simulink model "commhdlQPSKTxRxLoopback"  (R2025b)
settings: Solver=FixedStepDiscrete  StartTime=0.0  StopTime=0.03  RelTol=1e-3
PostLoadFcn:
  | hScopeConfig = get_param([gcs '/Receiver/QPSK Rx/Frequency and Time Synchronizer/Symbol Synchronizer/No HDL/QPSK Receiver Eye Diagram'],'ScopeConfiguration');
  | 
  | hScopeConfig.OpenAtSimulationStart = false;
  | hScopeConfig.Visible = false;
  | SamplesPerSymbol = 4;
  | %UpsamplesRx = 1;
  | clear hScopeConfig
InitFcn:
  | % RxAlign decoder latency (flat_simfix): 41 = netlist value used for HDL; set
  | % rxAlignLat = 25 in the base workspace before a model-level simulation.
  | if ~exist('rxAlignLat','var'), rxAlignLat = uint16(41); end
  | commhdlQPSKTxRxModelInit;
  | % Rate bridge: ADRV9002/Jupiter radio runs at 15.36 MHz = 2x the 7.68 MHz
  | % (4 samples/symbol @ Rsym=1.92 MHz) the QPSK Rx requires. The deployed
  | % Receiver must downsample the ADC stream by 2. UpsamplesRx=1 fed the QPSK
  | % Rx 8 sps (2x-upsampled) and broke symbol sync / the loopback bit check.
  | UpsamplesRx = 1;   %% T8 RATE FIX: rail 15.36e6 == ADC bus rate,
  | %% no ingress decimation (was 2 when the rail sat on the 7.68e6 rung)
  | UpsamplesTx = 1;
  | clear simTimingOffset;
StopFcn:
  | if exist('simTimingOffset','var')
  |   disp('Simulation completed');
  |   %QPSKTxRxVerification;
  | end
undefined symbols (not defined in the file or in its folder): Add, Config, fsym, randsrc, RandStream, Rsym, rxAlignLat, Shift
libraries: hdlsllib x141, simulink x45, dspsigops x30, dsphdlfiltering2 x6, dsphdlsigops2 x4, dsphdlmathfun2 x4, commdigbbndpm3 x4, dspmlti4 x2, commchan3 x1, commrflib2 x1, commcnvcod2 x1
(part 4 of 9)

== system commhdlQPSKTxRxLoopback/Transmitter/QPSK Tx/Bit Packetizer/Preamble Bits Generator ==
  activeFrame : Inport
  sampleCount : Inport  Port=2
  sampleCountValid : Inport  Port=3
  Compare To Constant2 : hdlsllib/Logic and Bit Operations/Compare To Constant  relop===  const=bitsPerPacket - 1  OutDataTypeStr=boolean
  Logical Operator3 : Logic  AllPortsSameDT=off  OutDataTypeStr=boolean
  Preamble Bits Store : Subsystem
  Unit Delay Enabled Synchronous : hdlsllib/Discrete/Unit Delay Enabled Synchronous  InitialCondition=0.0  SampleTime=-1
  preambleBits : Outport
  wires:
  sampleCount/1 -> Compare To Constant2/1, Preamble Bits Store/2(sampleCount)
  Logical Operator3/1 -> Unit Delay Enabled Synchronous/2
  Preamble Bits Store/1(preamble) -> preambleBits/1
  Compare To Constant2/1 -> Logical Operator3/1
  Unit Delay Enabled Synchronous/1 -> Preamble Bits Store/1(actualPreamble)
  sampleCountValid/1 -> Logical Operator3/2
  activeFrame/1 -> Unit Delay Enabled Synchronous/1

== system commhdlQPSKTxRxLoopback/TxRxComposite/Receiver/QPSK Rx/Automatic Gain Control ==
  dataIn : Inport
  validIn : Inport  Port=2
  agc_loop_gain : Inport  Port=3  OutDataTypeStr=uint32  SampleTime=1/(Rsym*SamplesPerSymbol)
  Data Type Conversion : DataTypeConversion  OutDataTypeStr=fixdt(1,16,10)  SaturateOnIntegerOverflow=off  RndMeth=Floor
  Delay{1..5} (5 alike) : Delay
  Error Detector : Subsystem
  Loop Filter : Subsystem
  Product : Product  OutDataTypeStr=Inherit: Same as first input
  dataOut : Outport
  validOut : Outport  Port=2
  wires:
  Product/1 -> Delay2/1
  Error Detector/1(err) -> Loop Filter/1(err)
  Delay1/1 -> Product/2
  Delay4/1 -> Product/1
  Delay3/1 -> validOut/1
  Delay2/1 -> dataOut/1, Error Detector/1(dataIn)
  Data Type Conversion/1 -> Delay1/1
  Loop Filter/1(gain) -> Data Type Conversion/1
  dataIn/1 -> Delay4/1
  Delay5/1 -> Delay3/1
  agc_loop_gain/1 -> Loop Filter/2(agc_loop_gain)
  validIn/1 -> Delay5/1

== system commhdlQPSKTxRxLoopback/TxRxComposite/Receiver/QPSK Rx/FEC Decoder Wrapper ==
  bitsIn : Inport
  startIn : Inport  Port=2
  endIn : Inport  Port=3
  validIn : Inport  Port=4
  skipCount : Inport  Port=5  OutDataTypeStr=uint32  SampleTime=1/(Rsym*SamplesPerSymbol)
  FecCapture : MATLAB Function  TreatAsAtomicUnit=on
  FecCounters : MATLAB Function  TreatAsAtomicUnit=on
  RxAlign : MATLAB Function  TreatAsAtomicUnit=on
  RxAlignLatency : Constant  Description=Decoder latency absorbed by RxAlign. rxAlignLat = 41 (netlist, default from InitFcn) or 25 (model simulation).  Value=rxAlignLat  OutDataTypeStr=uint16  SampleTime=Inf
  RxDeint : MATLAB Function  TreatAsAtomicUnit=on
  VitGate : Subsystem
  dataOut : Outport
  startOut : Outport  Port=2
  endOut : Outport  Port=3
  validOut : Outport  Port=4
  cnt_descr_in : Outport  Port=5
  cnt_frame_start : Outport  Port=6
  cnt_vit_reset : Outport  Port=7
  cnt_deint_valid : Outport  Port=8
  cnt_dec_bits : Outport  Port=9
  cnt_bist_start : Outport  Port=10
  cap_in : Outport  Port=11
  cap_deint : Outport  Port=12
  cap_out : Outport  Port=13
  wires:
  FecCounters/6(c6) -> cnt_bist_start/1
  FecCounters/3(c3) -> cnt_vit_reset/1
  FecCounters/2(c2) -> cnt_frame_start/1
  FecCapture/3(capOut) -> cap_out/1
  FecCapture/2(capDeint) -> cap_deint/1
  RxAlign/4(validOut) -> FecCapture/8(outValid), FecCounters/5(e5), validOut/1
  FecCapture/1(capIn) -> cap_in/1
  RxAlign/3(endOut) -> endOut/1
  bitsIn/1 -> RxDeint/1(dataIn), FecCapture/1(bitsIn)
  validIn/1 -> RxDeint/4(validIn), FecCounters/1(e1), FecCapture/2(validIn)
  FecCounters/5(c5) -> cnt_dec_bits/1
  startIn/1 -> RxDeint/2(startIn), FecCounters/2(e2), FecCapture/3(startIn)
  FecCounters/4(c4) -> cnt_deint_valid/1
  endIn/1 -> RxDeint/3(endIn)
  RxDeint/5(frameEnd) -> RxAlign/4(frameEnd)
  VitGate/1(decOut) -> RxAlign/1(decBit)
  RxDeint/1(codedPair) -> VitGate/1(pairIn), FecCapture/4(codedPair)
  FecCounters/1(c1) -> cnt_descr_in/1
  RxDeint/2(vitReset) -> VitGate/2(rstIn), FecCounters/3(e3)
  RxDeint/3(deintValid) -> VitGate/Enable, FecCounters/4(e4), RxAlign/2(deintValid), FecCapture/5(deintValid)
  skipCount/1 -> RxAlign/5(skipCount), FecCapture/7(skipCount)
  RxDeint/4(frameStart) -> RxAlign/3(frameStart)
  RxAlign/1(dataOut) -> FecCapture/6(decBit), dataOut/1
  RxAlign/2(startOut) -> FecCounters/6(e6), startOut/1
  RxAlignLatency/1 -> RxAlign/6(alignLat)

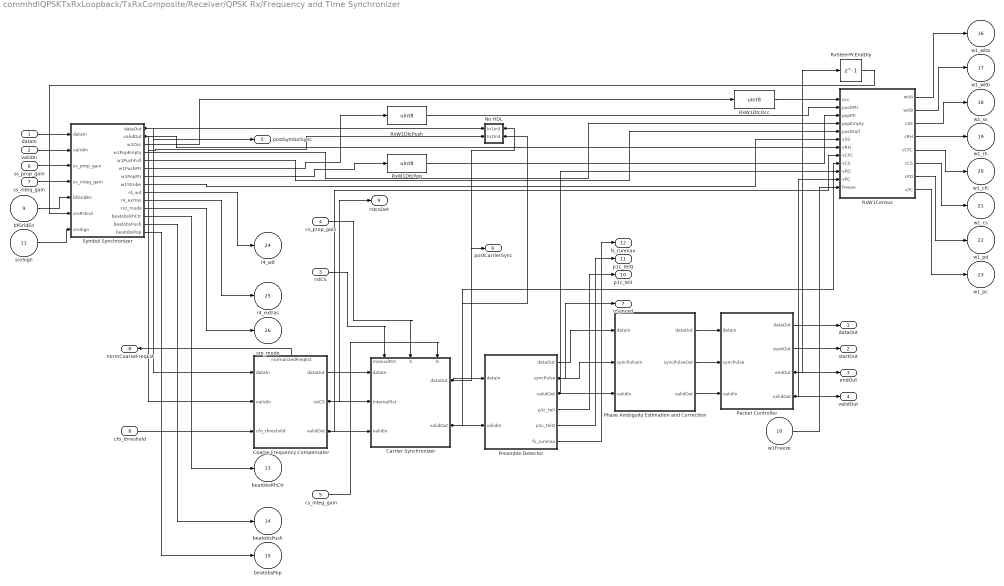
== system commhdlQPSKTxRxLoopback/TxRxComposite/Receiver/QPSK Rx/Frequency and Time Synchronizer ==
  dataIn : Inport
  validIn : Inport  Port=2
  rstCS : Inport  Port=3
  cs_prop_gain : Inport  Port=4  OutDataTypeStr=uint32  SampleTime=1/(Rsym*SamplesPerSymbol)
  cs_integ_gain : Inport  Port=5  OutDataTypeStr=uint32  SampleTime=1/(Rsym*SamplesPerSymbol)
  ss_prop_gain : Inport  Port=6  OutDataTypeStr=uint32  SampleTime=1/(Rsym*SamplesPerSymbol)
  ss_integ_gain : Inport  Port=7  OutDataTypeStr=uint32  SampleTime=1/(Rsym*SamplesPerSymbol)
  cfo_threshold : Inport  Port=8  OutDataTypeStr=uint32  SampleTime=1/(Rsym*SamplesPerSymbol)
  bfGridEn : Inport  Port=9  OutDataTypeStr=boolean
  w1Freeze : Inport  Port=10  OutDataTypeStr=boolean
  sroSign : Inport  Port=11  OutDataTypeStr=boolean
  Carrier Synchronizer : Subsystem
      settings: PortSchema="{\"entries\":[{\"content\":{\"sides\":[{\"content\":{\"connectorIds\":[\"In1\",\"In2\",\"In3\"]},\"type\":\"ConnectorPlacement.EquallySpacedRectSide\",\"uuid\":\"ee58e5dc-083a-48cb-b7f3-66ed8a15890f\"},{\"content\":{\"connectorIds\":[\"Out1\",\"Out2\"],\"side\":\"RIGHT\"},\"type\":\"ConnectorPlacement.EquallySpacedRectSide\",\"uuid\":\"6d121164-5065-4840-a82e-fa57a8e9650e\"},{\"content\":{\"connectorIds\":[\"In4\",\"In5\",\"In6\"],\"side\":\"TOP\"},\"type\":\"ConnectorPlacement.EquallySpacedRectSide\",\"uuid\":\"54d2b8e3-f516-4572-94a0-c914196ae8e4\"}]},\"type\":\"ConnectorPlacement.EquallySpacedConnector\",\"uuid\":\"0f2a6472-efd0-42ca-a030-ab436081b5e1\"}],\"packageUris\":[\"http://schema.mathworks.com/mf0/Connector/R2020b\"],\"version\":\"1.0\"}"
  Coarse Frequency Compensator : Subsystem
      settings: PortSchema="{\"entries\":[{\"content\":{\"sides\":[{\"content\":{\"connectorIds\":[\"In1\",\"In2\",\"In3\"]},\"type\":\"ConnectorPlacement.EquallySpacedRectSide\",\"uuid\":\"138aa5bd-62db-47d6-b55f-f529a6004434\"},{\"content\":{\"connectorIds\":[\"Out1\",\"Out2\",\"Out3\"],\"side\":\"RIGHT\"},\"type\":\"ConnectorPlacement.EquallySpacedRectSide\",\"uuid\":\"8e6ccec0-f736-48ab-be6d-feac886e083d\"},{\"content\":{\"connectorIds\":[\"Out4\"],\"side\":\"TOP\"},\"type\":\"ConnectorPlacement.EquallySpacedRectSide\",\"uuid\":\"d4535392-74fa-432a-a39c-b98ba26e8163\"},{\"content\":{\"side\":\"BOTTOM\"},\"type\":\"ConnectorPlacement.EquallySpacedRectSide\",\"uuid\":\"770ac6a2-7a02-4a77-858b-592982deaf6e\"}]},\"type\":\"ConnectorPlacement.EquallySpacedConnector\",\"uuid\":\"a9b944be-f88b-4ab6-a5e1-6824362eb9ca\"}],\"packageUris\":[\"http://schema.mathworks.com/mf0/Connector/R2020b\"],\"version\":\"1.0\"}"
  No HDL : Subsystem
      settings: PortSchema="{\"entries\":[{\"content\":{\"sides\":[{\"content\":{\"connectorIds\":[\"In1\",\"In2\"]},\"type\":\"ConnectorPlacement.EquallySpacedRectSide\",\"uuid\":\"df96a46d-149f-4580-adf6-e5cf26cffa9b\"},{\"content\":{\"connectorIds\":[\"In3\",\"In4\"],\"side\":\"RIGHT\"},\"type\":\"ConnectorPlacement.EquallySpacedRectSide\",\"uuid\":\"1c46d09c-cb37-4618-ac4e-e5ef50df41fb\"},{\"content\":{\"connectorIds\":[],\"side\":\"TOP\"},\"type\":\"ConnectorPlacement.EquallySpacedRectSide\",\"uuid\":\"7fe62300-46d7-4234-a31d-eecffed4f6e6\"},{\"content\":{\"connectorIds\":[],\"side\":\"BOTTOM\"},\"type\":\"ConnectorPlacement.EquallySpacedRectSide\",\"uuid\":\"05ecd563-28f5-4cfd-b718-5032a7458763\"}]},\"type\":\"ConnectorPlacement.EquallySpacedConnector\",\"uuid\":\"4b3d5859-a469-4389-9e5d-e5f07416a9a1\"}],\"packageUris\":[\"http://schema.mathworks.com/mf0/Connector/R2020b\"],\"version\":\"1.0\"}"
  Packet Controller : Subsystem
  Phase Ambiguity Estimation and Correction : Subsystem
  Preamble Detector : Subsystem
  RxSteerPcEndDly : Delay  DelayLength=1
  RxW1Census : MATLAB Function  TreatAsAtomicUnit=on
  RxW1DtcOcc : DataTypeConversion  OutDataTypeStr=uint8  ConvertRealWorld=Stored Integer (SI)  SaturateOnIntegerOverflow=off  RndMeth=Floor
  RxW1DtcPop : DataTypeConversion  OutDataTypeStr=uint8  ConvertRealWorld=Stored Integer (SI)  SaturateOnIntegerOverflow=off  RndMeth=Floor
  RxW1DtcPush : DataTypeConversion  OutDataTypeStr=uint8  ConvertRealWorld=Stored Integer (SI)  SaturateOnIntegerOverflow=off  RndMeth=Floor
  Symbol Synchronizer : Subsystem
  dataOut : Outport
  startOut : Outport  Port=2
  endOut : Outport  Port=3
  validOut : Outport  Port=4
  postSymbolSync : Outport  Port=5
  postCarrierSync : Outport  Port=6
  nSynced : Outport  Port=7
  normCoarseFreqEst : Outport  Port=8
  rstcsDet : Outport  Port=9
  p1c_telI : Outport  Port=10
  p1c_telQ : Outport  Port=11
  fs_runmax : Outport  Port=12
  beatobsRhCtr : Outport  Port=13
  beatobsPush : Outport  Port=14
  beatobsPop : Outport  Port=15
  w1_wita : Outport  Port=16
  w1_witb : Outport  Port=17
  w1_ss : Outport  Port=18
  w1_rh : Outport  Port=19
  w1_cfc : Outport  Port=20
  w1_cs : Outport  Port=21
  w1_pd : Outport  Port=22
  w1_pc : Outport  Port=23
  r4_wit : Outport  Port=24
  r4_extras : Outport  Port=25
  sro_mode : Outport  Port=26
  wires:
  RxW1Census/6(cCS) -> w1_cs/1
  RxSteerPcEndDly/1 -> Symbol Synchronizer/6(sroPcEnd)
  w1Freeze/1 -> RxW1Census/12(freeze)
  RxW1DtcOcc/1 -> RxW1Census/1(occ)
  Phase Ambiguity Estimation and Correction/2(syncPulseOut) -> Packet Controller/2(syncPulse)
  Phase Ambiguity Estimation and Correction/1(dataOut) -> Packet Controller/1(dataIn)
  RxW1Census/8(cPC) -> w1_pc/1
  Preamble Detector/6(fs_runmax) -> fs_runmax/1
  Preamble Detector/4(p1c_telI) -> p1c_telI/1
  Preamble Detector/1(dataOut) -> Phase Ambiguity Estimation and Correction/1(dataIn)
  RxW1DtcPush/1 -> RxW1Census/2(pushPtr)
  Symbol Synchronizer/7(w1PopPtr) -> RxW1DtcPop/1
  Symbol Synchronizer/5(w1PushFull) -> RxW1Census/5(pushFull)
  RxW1Census/1(witA) -> w1_wita/1
  cs_prop_gain/1 -> Carrier Synchronizer/5(cs_prop_gain)
  Symbol Synchronizer/4(w1PopEmpty) -> RxW1Census/4(popEmpty)
  RxW1Census/7(cPD) -> w1_pd/1
  Phase Ambiguity Estimation and Correction/3(validOut) -> Packet Controller/3(validIn)
  Symbol Synchronizer/2(validOut) -> Coarse Frequency Compensator/2(validIn), RxW1Census/7(vRH), No HDL/2(In2)
  Packet Controller/2(startOut) -> startOut/1
  sroSign/1 -> Symbol Synchronizer/7(sroSign)
  bfGridEn/1 -> Symbol Synchronizer/5(bfGridEn)
  Carrier Synchronizer/2(validOut) -> Preamble Detector/2(validIn), No HDL/4(In4), RxW1Census/9(vCS)
  cfo_threshold/1 -> Coarse Frequency Compensator/3(cfo_threshold)
  RxW1DtcPop/1 -> RxW1Census/3(popPtr)
  Symbol Synchronizer/3(w1Occ) -> RxW1DtcOcc/1
  RxW1Census/3(cSS) -> w1_ss/1
  Symbol Synchronizer/1(dataOut) -> postSymbolSync/1, Coarse Frequency Compensator/1(dataIn), No HDL/1(In1)
  Packet Controller/1(dataOut) -> dataOut/1
  ss_prop_gain/1 -> Symbol Synchronizer/3(ss_prop_gain)
  Symbol Synchronizer/6(w1PushPtr) -> RxW1DtcPush/1
  ss_integ_gain/1 -> Symbol Synchronizer/4(ss_integ_gain)
  Symbol Synchronizer/11(sro_mode) -> sro_mode/1
  Coarse Frequency Compensator/4(normalizedFreqEst) -> normCoarseFreqEst/1
  dataIn/1 -> Symbol Synchronizer/1(dataIn)
  Packet Controller/4(validOut) -> RxW1Census/11(vPC), validOut/1
  Symbol Synchronizer/9(r4_wit) -> r4_wit/1
  Preamble Detector/2(syncPulse) -> nSynced/1, Phase Ambiguity Estimation and Correction/2(syncPulseIn)
  Symbol Synchronizer/8(w1Strobe) -> RxW1Census/6(vSS)
  Symbol Synchronizer/13(beatobsPush) -> beatobsPush/1
  rstCS/1 -> Carrier Synchronizer/4(manualRst)
  Carrier Synchronizer/1(dataOut) -> postCarrierSync/1, Preamble Detector/1(dataIn), No HDL/3(In3)
  Symbol Synchronizer/10(r4_extras) -> r4_extras/1
  Preamble Detector/5(p1c_telQ) -> p1c_telQ/1
  Symbol Synchronizer/12(beatobsRhCtr) -> beatobsRhCtr/1
  Coarse Frequency Compensator/1(dataOut) -> Carrier Synchronizer/1(dataIn)
  Symbol Synchronizer/14(beatobsPop) -> beatobsPop/1
  RxW1Census/4(cRH) -> w1_rh/1
  Coarse Frequency Compensator/3(validOut) -> Carrier Synchronizer/3(validIn), RxW1Census/8(vCFC)
  RxW1Census/2(witB) -> w1_witb/1
  validIn/1 -> Symbol Synchronizer/2(validIn)
  Coarse Frequency Compensator/2(rstCS) -> rstcsDet/1, Carrier Synchronizer/2(internalRst)
  RxW1Census/5(cCFC) -> w1_cfc/1
  Packet Controller/3(endOut) -> RxSteerPcEndDly/1, endOut/1
  Preamble Detector/3(validOut) -> Phase Ambiguity Estimation and Correction/3(validIn), RxW1Census/10(vPD)
  cs_integ_gain/1 -> Carrier Synchronizer/6(cs_integ_gain)

== system commhdlQPSKTxRxLoopback/TxRxComposite/Receiver/QPSK Rx/QPSK Demodulator ==
  dataIn : Inport
  startIn : Inport  Port=2
  endIn : Inport  Port=3
  validIn : Inport  Port=4
  bfSerEn : Inport  Port=5  OutDataTypeStr=boolean
  BfSerAnd : Logic  AllPortsSameDT=off  OutDataTypeStr=boolean
  Delay{,1..13} (14 alike) : Delay  DelayLength=1
  QPSK Demodulator Baseband : commdigbbndpm3/QPSK Demodulator Baseband  OutType=Bit  DecType=Hard decision  VarSource=Dialog  Variance=1  Dec=Gray  Ph=pi/4  outDtype1=boolean  outDtype2=Inherit via internal rule  derotateFactorWordLen=16  derotateFactorDataTypeStr=Inherit: Same word length as input  derotateFactorLastDataTypeStr=Inherit: Same word length as input
  Serializer : Subsystem
  Signal Specification : SignalSpecification  Dimensions=1
  dataOut : Outport
  startOut : Outport  Port=2
  endOut : Outport  Port=3
  validOut : Outport  Port=4
  beatobsDecis : Outport  Port=5
  wires:
  Delay10/1 -> startOut/1
  Delay8/1 -> dataOut/1
  Delay4/1 -> Delay10/1
  Delay6/1 -> Delay4/1
  Serializer/2(Out2) -> Delay9/1
  Serializer/1(Out1) -> Delay8/1
  Delay9/1 -> validOut/1
  Delay2/1 -> Delay6/1
  endIn/1 -> Delay3/1
  Delay13/1 -> Delay11/1
  Delay12/1 -> Serializer/1(u)
  startIn/1 -> BfSerAnd/1, Delay2/1
  Delay3/1 -> Delay7/1
  Signal Specification/1 -> Delay/1
  dataIn/1 -> Signal Specification/1
  Delay7/1 -> Delay13/1
  Delay/1 -> QPSK Demodulator Baseband/1
  validIn/1 -> Delay1/1
  BfSerAnd/1 -> Serializer/3(bfAnchor)
  QPSK Demodulator Baseband/1 -> beatobsDecis/1, Delay12/1
  Delay1/1 -> Delay5/1
  Delay5/1 -> Serializer/2(In2)
  bfSerEn/1 -> BfSerAnd/2
  Delay11/1 -> endOut/1

== system commhdlQPSKTxRxLoopback/TxRxComposite/Transmitter/Input Data/FEC Tx Encoder K5 ==
  bitIn : Inport
  enable : Inport  Port=2
  reset : Inport  Port=3
  start : Inport  Port=4
  ConvEncK5 : MATLAB Function  TreatAsAtomicUnit=on
  TxGateK5 : MATLAB Function  TreatAsAtomicUnit=on
  TxInterleaveK5 : MATLAB Function  TreatAsAtomicUnit=on
  encBit : Outport
  wires:
  TxInterleaveK5/1(dataOut) -> encBit/1
  ConvEncK5/1(codedPair) -> TxInterleaveK5/1(codedPair)
  TxGateK5/4(beatIdx) -> TxInterleaveK5/3(beatIdx)
  TxGateK5/2(encReset) -> ConvEncK5/2(encReset)
  TxGateK5/1(infoBit) -> ConvEncK5/1(infoBit)
  TxGateK5/6(frameStart) -> TxInterleaveK5/5(frameStart)
  TxGateK5/3(infoValid) -> ConvEncK5/3(infoValid), TxInterleaveK5/2(infoValid)
  reset/1 -> TxGateK5/3(reset)
  enable/1 -> TxGateK5/2(enable)
  TxGateK5/5(frameValid) -> TxInterleaveK5/4(frameValid)
  start/1 -> TxGateK5/4(start)
  bitIn/1 -> TxGateK5/1(bitIn)

== system commhdlQPSKTxRxLoopback/TxRxComposite/Transmitter/Input Data/Message Generator ==
  reset : Inport
  enable : Inport  Port=2
  MATLAB Function : MATLAB Function  TreatAsAtomicUnit=on
  out : Outport
  stop : Outport  Port=2
  start : Outport  Port=3
  valid : Outport  Port=4
  count : Outport  Port=5
  msg_count_out : Outport  Port=6
  wires:
  MATLAB Function/6(msg_count_out) -> msg_count_out/1
  MATLAB Function/5(count_out) -> count/1
  MATLAB Function/4(valid) -> valid/1
  MATLAB Function/3(stop) -> stop/1
  MATLAB Function/2(start) -> start/1
  MATLAB Function/1(out) -> out/1
  reset/1 -> MATLAB Function/2(reset)
  enable/1 -> MATLAB Function/1(enable)

== system commhdlQPSKTxRxLoopback/TxRxComposite/Transmitter/QPSK Tx/Bit Packetizer ==
  dataIn : Inport
  validIn : Inport  Port=2
  Compare To Constant : hdlsllib/Logic and Bit Operations/Compare To Constant  relop===  const=length(Preamble)  OutDataTypeStr=boolean
  Compare To Constant1 : hdlsllib/Logic and Bit Operations/Compare To Constant  relop===  const=bitsPerPacket - 1  OutDataTypeStr=boolean
  Compare To Constant2 : hdlsllib/Logic and Bit Operations/Compare To Constant  relop=>=  const=length(Preamble)  OutDataTypeStr=boolean
  Data Bits FIFO : Subsystem
  Data Type Conversion : DataTypeConversion  OutDataTypeStr=boolean  SaturateOnIntegerOverflow=off  RndMeth=Floor
  DataReadyPaceCmp : simulink/Logic and Bit Operations/Compare To Constant  relop=>=  const=SamplesPerSymbol/2 - 1  OutDataTypeStr=boolean
  HDL Counter : hdlsllib/Sources/HDL Counter  CountType=Count limited  CountInit=0  CountStep=1  CountMax=max(1, SamplesPerSymbol/2 - 1)  CountFromType=Initial value  CountFrom=0  CountResetPort=off  CountLoadPort=off  CountEnbPort=on  CountDirPort=off  CountHitOutputPort=off  CountDataType=Unsigned  CountWordLen=max(1, nextpow2(SamplesPerSymbol/2))  CountFracLen=0  CountSampTime=1
  Logical Operator : Logic  AllPortsSameDT=off  OutDataTypeStr=boolean
  Logical Operator1 : Logic  AllPortsSameDT=off  OutDataTypeStr=boolean
  Logical Operator2 : Logic  Operator=NOT  AllPortsSameDT=off  OutDataTypeStr=boolean
  Preamble Bits Generator : Subsystem
  Switch : Switch  Criteria=u2 ~= 0  SaturateOnIntegerOverflow=off  InputSameDT=off
  TxF3ReadyGate : Logic  AllPortsSameDT=off  OutDataTypeStr=boolean
  bitsOut : Outport
  dataStart : Outport  Port=2
  dataEnd : Outport  Port=3
  bitsValid : Outport  Port=4
  dataReady : Outport  Port=5
  wires:
  TxF3ReadyGate/1 -> Data Type Conversion/1
  DataReadyPaceCmp/1 -> TxF3ReadyGate/1
  Logical Operator1/1 -> dataEnd/1
  Logical Operator/1 -> dataStart/1
  validIn/1 -> Data Bits FIFO/2(push)
  Data Bits FIFO/1(dataOut) -> Switch/1
  Logical Operator2/1 -> HDL Counter/1, TxF3ReadyGate/2
  Data Bits FIFO/2(activeFrame) -> Preamble Bits Generator/1(activeFrame)
  HDL Counter/1 -> DataReadyPaceCmp/1
  Data Bits FIFO/4(sampleCountValid) -> Preamble Bits Generator/3(sampleCountValid), bitsValid/1, Logical Operator/2, Logical Operator1/1
  Data Type Conversion/1 -> dataReady/1
  Data Bits FIFO/5(fullRAM) -> Logical Operator2/1
  dataIn/1 -> Data Bits FIFO/1(data)
  Compare To Constant2/1 -> Switch/2
  Preamble Bits Generator/1(preambleBits) -> Switch/3
  Data Bits FIFO/3(sampleCount) -> Preamble Bits Generator/2(sampleCount), Compare To Constant1/1, Compare To Constant/1, Compare To Constant2/1
  Compare To Constant/1 -> Logical Operator/1
  Compare To Constant1/1 -> Logical Operator1/2
  Switch/1 -> bitsOut/1

== system commhdlQPSKTxRxLoopback/TxRxComposite/Transmitter/QPSK Tx/HDL Data Scrambler ==
  note: HDL Data Scrambler
      | Polynomial: x^7+x^4+1
      | Initial state: [1 0 1 1 1 0 1]
  dataIn : Inport
  startIn : Inport  Port=2
  endIn : Inport  Port=3
  validIn : Inport  Port=4
  BIT_XOR : Logic  Operator=XOR  IconShape=distinctive  AllPortsSameDT=off  OutDataTypeStr=boolean
  BIT_XOR2 : Logic  Operator=XOR  IconShape=distinctive  AllPortsSameDT=off  OutDataTypeStr=boolean
  Delay{,1,3..4} (4 alike) : Delay  DelayLength=1
  EnableScrambling : Constant  Value=false  SampleTime=-1
  Logical Operator : Logic  IconShape=distinctive  AllPortsSameDT=off  OutDataTypeStr=boolean
  Switch : Switch  Criteria=u2 > Threshold  SaturateOnIntegerOverflow=off  InputSameDT=off
  Unit Delay Enabled Resettable Synchronous{,2..3,5,7} (5 alike) : hdlsllib/Discrete/Unit Delay Enabled Resettable Synchronous  InitialCondition=1  SampleTime=-1
  Unit Delay Enabled Resettable Synchronous1 : hdlsllib/Discrete/Unit Delay Enabled Resettable Synchronous  InitialCondition=0  SampleTime=-1
  Unit Delay Enabled Resettable Synchronous4 : hdlsllib/Discrete/Unit Delay Enabled Resettable Synchronous  InitialCondition=0  SampleTime=-1
  Unit Delay Enabled Resettable Synchronous6 : hdlsllib/Discrete/Unit Delay Enabled Resettable Synchronous  InitialCondition=0.0  SampleTime=-1
  dataOut : Outport  InitialOutput=0
  validOut : Outport  Port=2  InitialOutput=0
  wires:
  Delay3/1 -> dataOut/1
  BIT_XOR2/1 -> Switch/1
  Logical Operator/1 -> BIT_XOR2/2
  Delay4/1 -> validOut/1
  Unit Delay Enabled Resettable Synchronous4/1 -> Logical Operator/1
  Unit Delay Enabled Resettable Synchronous7/1 -> BIT_XOR/1
  Delay/1 -> BIT_XOR2/1, Switch/3
  Unit Delay Enabled Resettable Synchronous5/1 -> Unit Delay Enabled Resettable Synchronous6/1
  dataIn/1 -> Delay/1
  Unit Delay Enabled Resettable Synchronous3/1 -> BIT_XOR/2, Unit Delay Enabled Resettable Synchronous5/1
  Unit Delay Enabled Resettable Synchronous2/1 -> Unit Delay Enabled Resettable Synchronous3/1
  Unit Delay Enabled Resettable Synchronous1/1 -> Unit Delay Enabled Resettable Synchronous2/1
  Unit Delay Enabled Resettable Synchronous/1 -> Unit Delay Enabled Resettable Synchronous1/1
  Switch/1 -> Delay3/1
  startIn/1 -> Unit Delay Enabled Resettable Synchronous4/1, Unit Delay Enabled Resettable Synchronous4/2, Unit Delay Enabled Resettable Synchronous7/3, Unit Delay Enabled Resettable Synchronous6/3, Unit Delay Enabled Resettable Synchronous1/3, Unit Delay Enabled Resettable Synchronous2/3, Unit Delay Enabled Resettable Synchronous/3, Unit Delay Enabled Resettable Synchronous5/3, Unit Delay Enabled Resettable Synchronous3/3
  EnableScrambling/1 -> Switch/2
  validIn/1 -> Delay1/1
  Unit Delay Enabled Resettable Synchronous6/1 -> Unit Delay Enabled Resettable Synchronous7/1
  endIn/1 -> Unit Delay Enabled Resettable Synchronous4/3
  Delay1/1 -> Delay4/1, Unit Delay Enabled Resettable Synchronous6/2, Unit Delay Enabled Resettable Synchronous3/2, Unit Delay Enabled Resettable Synchronous7/2, Unit Delay Enabled Resettable Synchronous1/2, Unit Delay Enabled Resettable Synchronous/2, Unit Delay Enabled Resettable Synchronous5/2, Unit Delay Enabled Resettable Synchronous2/2
  BIT_XOR/1 -> Logical Operator/2, Unit Delay Enabled Resettable Synchronous/1

== system commhdlQPSKTxRxLoopback/TxRxComposite/Transmitter/QPSK Tx/QPSK Modulator ==
  dataIn : Inport
  validIn : Inport  Port=2
  Compare To Constant : simulink/Logic and Bit Operations/Compare To Constant  relop===  const=0  OutDataTypeStr=boolean
  Compare To Constant1 : simulink/Logic and Bit Operations/Compare To Constant  relop===  const=1  OutDataTypeStr=boolean
  Delay{,1..5,11..12} (8 alike) : Delay  DelayLength=1
  HDL Counter : hdlsllib/Sources/HDL Counter  CountType=Count limited  CountInit=0  CountStep=1  CountMax=1  CountFromType=Initial value  CountFrom=0  CountResetPort=off  CountLoadPort=off  CountEnbPort=on  CountDirPort=off  CountHitOutputPort=off  CountDataType=Unsigned  CountWordLen=1  CountFracLen=0  CountSampTime=1
  Logical Operator : Logic  IconShape=distinctive  AllPortsSameDT=off  OutDataTypeStr=boolean
  Logical Operator1 : Logic  IconShape=distinctive  AllPortsSameDT=off  OutDataTypeStr=boolean
  Mux : Mux  Inputs=2
  Null : Constant  Value=complex(0,0)  OutDataTypeStr=fixdt(1,16,15)  SampleTime=1/(Rsym*SamplesPerSymbol)
  QPSK Modulator Baseband : commdigbbndpm3/QPSK Modulator Baseband  InType=Bit  Enc=Gray  Ph=pi/4  outDtype=Fixed-point  outWordLen=16  outUDDataType=sfix(16)  outFracLenMode=User-defined  outFracLen=15  outDataTypeStr=fixdt(1,16,15)  outLastDataTypeStr=fixdt(1,16,15)
  Switch3 : Switch  Threshold=1  SaturateOnIntegerOverflow=off  InputSameDT=off
  Unit Delay Enabled Synchronous : hdlsllib/Discrete/Unit Delay Enabled Synchronous  InitialCondition=0.0  SampleTime=-1
  dataOut : Outport
  validOut : Outport  Port=2
  wires:
  Delay2/1 -> dataOut/1
  Switch3/1 -> Delay2/1
  Null/1 -> Switch3/3
  QPSK Modulator Baseband/1 -> Delay11/1
  Delay4/1 -> QPSK Modulator Baseband/1
  validIn/1 -> Delay1/1
  Unit Delay Enabled Synchronous/1 -> Mux/1
  Delay1/1 -> HDL Counter/1, Logical Operator/1, Logical Operator1/2
  dataIn/1 -> Delay/1
  Logical Operator1/1 -> Delay5/1
  HDL Counter/1 -> Compare To Constant/1, Compare To Constant1/1
  Compare To Constant/1 -> Logical Operator/2
  Delay3/1 -> validOut/1
  Compare To Constant1/1 -> Logical Operator1/1
  Delay/1 -> Unit Delay Enabled Synchronous/1, Mux/2
  Logical Operator/1 -> Unit Delay Enabled Synchronous/2
  Delay11/1 -> Switch3/1
  Delay12/1 -> Delay3/1, Switch3/2
  Delay5/1 -> Delay12/1
  Mux/1 -> Delay4/1

== system commhdlQPSKTxRxLoopback/TxRxComposite/Transmitter/QPSK Tx/RRC Transmit Filter ==
  dataIn : Inport
  validIn : Inport  Port=2
  Data Type Conversion : DataTypeConversion  OutDataTypeStr=fixdt(1,17,16)  SaturateOnIntegerOverflow=off  RndMeth=Floor
  Data Type Conversion1 : DataTypeConversion  OutDataTypeStr=fixdt(1,16,14)  SaturateOnIntegerOverflow=off  RndMeth=Floor
  Delay1 : Delay  DelayLength=1
  Delay2 : Delay  DelayLength=1
  Delay3 : Delay  DelayLength=1
  RRC Filter : dsphdlfiltering2/Discrete FIR Filter  NumeratorSource=Property  Numerator=RRCCoef  NumeratorPrototype=[]  FilterStructure=Direct form systolic  SerializationOption=Minimum number of cycles between valid input samples  NumCycles=2  NumberOfMultipliers=2  SimulateUsing=Code generation  roundingMode=Floor  overflowMode=off  CoefficientsDataTypeStr=Inherit: Same word length as input  OutputDataTypeStr=Inherit: Same word length as input  ResetInputPort=off  HDLGlobalReset=off  CoeffMultiplier=Multiplier  UseMultForPow2Coeff=on  FrameInputSymmOptim=off
  Unit Delay Enabled Synchronous1 : hdlsllib/Discrete/Unit Delay Enabled Synchronous  InitialCondition=0  SampleTime=-1
  dataOut : Outport
  validOut : Outport  Port=2
  wires:
  Delay1/1 -> dataOut/1
  Delay2/1 -> validOut/1
  RRC Filter/2 -> Delay2/1
  RRC Filter/1 -> Data Type Conversion1/1
  Delay3/1 -> RRC Filter/1
  Unit Delay Enabled Synchronous1/1 -> RRC Filter/2
  validIn/1 -> Unit Delay Enabled Synchronous1/2, Unit Delay Enabled Synchronous1/1
  Data Type Conversion1/1 -> Delay1/1
  Data Type Conversion/1 -> Delay3/1
  dataIn/1 -> Data Type Conversion/1

== system commhdlQPSKTxRxLoopback/Receiver/QPSK Rx/Frequency and Time Synchronizer/Carrier Synchronizer/Direct Digital Synthesis ==
  rst : Inport
  validIn : Inport  Port=2
  phaseInc : Inport  Port=3
  Data Type Conversion : DataTypeConversion  OutDataTypeStr=fixdt(1,21,21)  SaturateOnIntegerOverflow=off  RndMeth=Floor
  Data Type Conversion1 : DataTypeConversion  OutDataTypeStr=fixdt(1,21,0)  ConvertRealWorld=Stored Integer (SI)  SaturateOnIntegerOverflow=off  RndMeth=Floor
  Delay : Delay  DelayLength=1
  NCO : dsphdlsigops2/NCO  PhaseIncrementSource=Input port  PhaseIncrement=0  PhaseOffsetSource=Property  PhaseOffset=0  DitherSource=Property  NumDitherBits=11  SamplesPerFrame=1  LUTCompress=off  ResetAction=on  Waveform=Complex exponential  PhasePort=off  SimulateUsing=Code generation  AccumulatorWL=21  PhaseQuantization=on  NumQuantizerAccumulatorBits=14  OutputDataType=Binary point scaling  OutputWL=16  OutputFL=14
  Terminator : Terminator
  expOut : Outport
  wires:
  Data Type Conversion/1 -> Data Type Conversion1/1
  NCO/1 -> expOut/1
  validIn/1 -> NCO/3
  Data Type Conversion1/1 -> NCO/1
  NCO/2 -> Terminator/1
  Delay/1 -> Data Type Conversion/1
  phaseInc/1 -> Delay/1
  rst/1 -> NCO/2

== system commhdlQPSKTxRxLoopback/Receiver/QPSK Rx/Frequency and Time Synchronizer/Carrier Synchronizer/Loop Filter ==
  e : Inport
  validIn : Inport  Port=2
  internalRst : Inport  Port=3
  externalRst : Inport  Port=4
  Add : Sum  Inputs=+|+
  Add1 : Sum  Inputs=|++  OutDataTypeStr=Inherit: Same as first input
  Data Type Conversion1 : DataTypeConversion  OutDataTypeStr=fixdt(1,29,29)  SaturateOnIntegerOverflow=off  RndMeth=Floor
  Data Type Conversion2 : DataTypeConversion  OutDataTypeStr=fixdt(1,39,39)  SaturateOnIntegerOverflow=off  RndMeth=Floor
  Delay : Delay  DelayLength=1
  Delay{1..11,13} (12 alike) : Delay
  Delay12 : Delay  DelayLength=1
  Gain : Gain  Gain=fi(CSLoopFilterIntegGain/(2*pi),0,16,16)  ParamDataTypeStr=Inherit: Inherit from 'Gain'
  Gain1 : Gain  Gain=fi(CSLoopFilterPropGain/(2*pi),0,16,16)  ParamDataTypeStr=Inherit: Inherit from 'Gain'
  Logical Operator : Logic  Operator=OR  AllPortsSameDT=off  OutDataTypeStr=boolean
  Unit Delay Enabled Resettable Synchronous : hdlsllib/Discrete/Unit Delay Enabled Resettable Synchronous  InitialCondition=0.0  SampleTime=-1
  Unit Delay Enabled Resettable Synchronous1 : hdlsllib/Discrete/Unit Delay Enabled Resettable Synchronous  InitialCondition=0.0  SampleTime=-1
  v : Outport
  valid : Outport  Port=2
  rst : Outport  Port=3
  wires:
  Delay6/1 -> Data Type Conversion1/1
  Delay5/1 -> Gain/1
  Delay7/1 -> Gain1/1
  Gain/1 -> Delay1/1
  Data Type Conversion2/1 -> Add1/1
  Delay3/1 -> Add/2
  Delay1/1 -> Data Type Conversion2/1
  Gain1/1 -> Delay6/1
  Delay2/1 -> Add/1
  Add/1 -> v/1
  e/1 -> Delay7/1, Delay5/1
  Data Type Conversion1/1 -> Unit Delay Enabled Resettable Synchronous/1
  Add1/1 -> Unit Delay Enabled Resettable Synchronous1/1
  Unit Delay Enabled Resettable Synchronous1/1 -> Delay3/1, Add1/2
  Unit Delay Enabled Resettable Synchronous/1 -> Delay2/1
  Logical Operator/1 -> Unit Delay Enabled Resettable Synchronous/3, Unit Delay Enabled Resettable Synchronous1/3
  validIn/1 -> Delay8/1
  Delay8/1 -> Delay4/1
  externalRst/1 -> Logical Operator/1
  internalRst/1 -> Delay9/1
  Delay9/1 -> Delay10/1
  Delay10/1 -> Delay12/1, Logical Operator/2
  Delay4/1 -> Unit Delay Enabled Resettable Synchronous/2, Unit Delay Enabled Resettable Synchronous1/2, Delay/1
  Delay11/1 -> valid/1
  Delay/1 -> Delay11/1
  Delay12/1 -> Delay13/1
  Delay13/1 -> rst/1

== system commhdlQPSKTxRxLoopback/Receiver/QPSK Rx/Frequency and Time Synchronizer/Carrier Synchronizer/Phase Error Detector ==
  dataIn : Inport
  Add : Sum  Inputs=+|-
  Compare To Constant : simulink/Logic and Bit Operations/Compare To Constant  relop=>=  const=0  OutDataTypeStr=boolean
  Compare To Constant1 : simulink/Logic and Bit Operations/Compare To Constant  relop=>=  const=0  OutDataTypeStr=boolean
  Complex to Real-Imag : ComplexToRealImag
  Constant : Constant  OutDataTypeStr=fixdt(1,2,0)  SampleTime=1/(Rsym*SamplesPerSymbol)
  Constant1 : Constant  Value=-1  OutDataTypeStr=fixdt(1,2,0)  SampleTime=1/(Rsym*SamplesPerSymbol)
  Constant2 : Constant  OutDataTypeStr=fixdt(1,2,0)  SampleTime=1/(Rsym*SamplesPerSymbol)
  Constant3 : Constant  Value=-1  OutDataTypeStr=fixdt(1,2,0)  SampleTime=1/(Rsym*SamplesPerSymbol)
  Data Type Conversion3 : DataTypeConversion  OutDataTypeStr=fixdt(1,10+3,10)  SaturateOnIntegerOverflow=off  RndMeth=Floor
  Delay{,1..6} (7 alike) : Delay
  Product : Product
  Product1 : Product
  Switch : Switch  Threshold=1  SaturateOnIntegerOverflow=off  InputSameDT=off
  Switch1 : Switch  Threshold=1  SaturateOnIntegerOverflow=off  InputSameDT=off
  PhaseError : Outport
  wires:
  Complex to Real-Imag/1 -> Delay2/1, Compare To Constant/1
  Compare To Constant1/1 -> Switch1/2
  Constant/1 -> Switch/1
  Constant3/1 -> Switch1/3
  Constant2/1 -> Switch1/1
  Constant1/1 -> Switch/3
  Compare To Constant/1 -> Switch/2
  Add/1 -> Delay6/1
  Switch/1 -> Delay/1
  Product1/1 -> Delay5/1
  Product/1 -> Delay4/1
  Switch1/1 -> Delay3/1
  Complex to Real-Imag/2 -> Delay1/1, Compare To Constant1/1
  dataIn/1 -> Complex to Real-Imag/1
  Delay/1 -> Product/1
  Delay1/1 -> Product/2
  Delay2/1 -> Product1/1
  Delay3/1 -> Product1/2
  Delay4/1 -> Add/1
  Delay5/1 -> Add/2
  Delay6/1 -> Data Type Conversion3/1
  Data Type Conversion3/1 -> PhaseError/1

== system commhdlQPSKTxRxLoopback/Receiver/QPSK Rx/Frequency and Time Synchronizer/Coarse Frequency Compensator/CFO step change detector ==
  note: fixed point precision loss warning supressed for this subsystem
  In1 : Inport
  Add : Sum  Inputs=+-
  Compare To Constant : simulink/Logic and Bit Operations/Compare To Constant  relop=>  const=fi(CFOChangeDetectThreshold,1,22,21)  OutDataTypeStr=boolean
  Compare To Constant1 : simulink/Logic and Bit Operations/Compare To Constant  relop=<  const=fi(-CFOChangeDetectThreshold,1,22,21)  OutDataTypeStr=boolean
  Delay : Delay  DelayLength=6
  Delay1 : Delay  DelayLength=1
  Logical Operator : Logic  Operator=OR  AllPortsSameDT=off  OutDataTypeStr=boolean
  Out1 : Outport
  wires:
  In1/1 -> Add/1, Delay1/1
  Delay/1 -> Out1/1
  Delay1/1 -> Add/2
  Add/1 -> Compare To Constant/1, Compare To Constant1/1
  Compare To Constant/1 -> Logical Operator/1
  Logical Operator/1 -> Delay/1
  Compare To Constant1/1 -> Logical Operator/2

== system commhdlQPSKTxRxLoopback/Receiver/QPSK Rx/Frequency and Time Synchronizer/Coarse Frequency Compensator/Coarse Frequency Estimator ==
  dataIn : Inport
  validIn : Inport  Port=2
  Delay{1,9..12} (5 alike) : Delay  DelayLength=1
  Delay{2..8} (7 alike) : Delay
  Extract Frequency : Subsystem
  Gain1 : Gain  Gain=1/integAvgLen  ParamDataTypeStr=fixdt(0,nextpow2(integAvgLen),nextpow2(integAvgLen))  OutDataTypeStr=Inherit: Same as input
  Integrator : Subsystem
  Math Function : Math  Operator=conj
  Product : Product
  Unit Delay Enabled Synchronous : hdlsllib/Discrete/Unit Delay Enabled Synchronous  InitialCondition=0.0  SampleTime=-1
  normFreqEst : Outport
  wires:
  Delay8/1 -> Product/2
  Delay7/1 -> Product/1
  Delay6/1 -> Delay3/1
  Delay4/1 -> Integrator/2(validIn)
  Delay2/1 -> Integrator/1(dataIn)
  Delay1/1 -> Delay7/1
  Unit Delay Enabled Synchronous/1 -> Delay12/1
  Delay9/1 -> Delay6/1
  Delay3/1 -> Delay4/1
  Delay5/1 -> Gain1/1
  Gain1/1 -> Delay2/1
  Product/1 -> Delay5/1
  Math Function/1 -> Delay8/1
  Delay10/1 -> Extract Frequency/1(datain)
  Delay11/1 -> Extract Frequency/2(validIn)
  Integrator/1(IntegOut) -> Delay10/1
  Integrator/2(IntegValid) -> Delay11/1
  Extract Frequency/1(normFreqOut) -> normFreqEst/1
  dataIn/1 -> Delay1/1, Unit Delay Enabled Synchronous/1
  validIn/1 -> Unit Delay Enabled Synchronous/2, Delay9/1
  Delay12/1 -> Math Function/1

== system commhdlQPSKTxRxLoopback/Receiver/QPSK Rx/Frequency and Time Synchronizer/Coarse Frequency Compensator/Raise Power to 4 ==
  dataIn : Inport
  validIn : Inport  Port=2
  Delay{1..8,11..12} (10 alike) : Delay
  Delay10 : Delay  DelayLength=1
  Delay9 : Delay  DelayLength=1
  Product1 : Product  OutDataTypeStr=Inherit: Same as first input
  Product2 : Product  OutDataTypeStr=Inherit: Same as first input
  dataOut : Outport
  validOut : Outport  Port=2
  wires:
  Delay12/1 -> validOut/1
  Delay11/1 -> dataOut/1
  Delay10/1 -> Delay8/1
  Delay9/1 -> Delay6/1, Delay7/1
  Delay8/1 -> Delay12/1
  Delay7/1 -> Product2/2
  Delay6/1 -> Product2/1
  Delay5/1 -> Delay2/1
  Delay4/1 -> Product1/2
  Delay3/1 -> Product1/1
  validIn/1 -> Delay5/1
  Product2/1 -> Delay11/1
  Delay2/1 -> Delay10/1
  Product1/1 -> Delay1/1
  Delay1/1 -> Delay9/1
  dataIn/1 -> Delay4/1, Delay3/1

== system commhdlQPSKTxRxLoopback/Receiver/QPSK Rx/Frequency and Time Synchronizer/No HDL/Subsystem ==
  In1 : Inport
  Enable : EnablePort
  To Workspace : ToWorkspace  VariableName=simAfterCS  SampleTime=-1
      settings: Save2DSignal=2-D array (concatenate along first dimension)
  wires:
  In1/1 -> To Workspace/1

== system commhdlQPSKTxRxLoopback/Receiver/QPSK Rx/Frequency and Time Synchronizer/Packet Controller/End Generator ==
  validIn : Inport
  rst : Inport  Port=2
  Compare To Constant : simulink/Logic and Bit Operations/Compare To Constant  relop===  const=1120-1  OutDataTypeStr=boolean
  Delay6 : Delay  DelayLength=1
  HDL Counter : hdlsllib/Sources/HDL Counter  CountType=Count limited  CountInit=0  CountStep=1  CountMax=1120 -1  CountFromType=Initial value  CountFrom=0  CountResetPort=on  CountLoadPort=off  CountEnbPort=on  CountDirPort=off  CountHitOutputPort=off  CountDataType=Unsigned  CountWordLen=nextpow2(1120-1)  CountFracLen=0  CountSampTime=1
  Logical Operator1 : Logic  IconShape=distinctive  AllPortsSameDT=off  OutDataTypeStr=boolean
  endOut : Outport
  wires:
  Compare To Constant/1 -> Logical Operator1/1
  HDL Counter/1 -> Compare To Constant/1
  validIn/1 -> HDL Counter/2, Logical Operator1/2
  rst/1 -> HDL Counter/1
  Logical Operator1/1 -> Delay6/1
  Delay6/1 -> endOut/1

== system commhdlQPSKTxRxLoopback/Receiver/QPSK Rx/Frequency and Time Synchronizer/Phase Ambiguity Estimation and Correction/Average Estimates ==
  endIn : Inport
  estin : Inport  Port=2
  validIn : Inport  Port=3
  Add : Sum  Inputs=++|
  Data Type Conversion : DataTypeConversion  OutDataTypeStr=fixdt(1,16+8,13)  SaturateOnIntegerOverflow=off  RndMeth=Floor
  Data Type Conversion1 : DataTypeConversion  OutDataTypeStr=fixdt(1,16+8,13)  SaturateOnIntegerOverflow=off  RndMeth=Floor
  Data Type Conversion2 : DataTypeConversion  OutDataTypeStr=fixdt(1,16,14)  SaturateOnIntegerOverflow=off  RndMeth=Floor
  Delay{,1..3} (4 alike) : Delay  DelayLength=1
  Divide by 8 : DataTypeConversion  OutDataTypeStr=fixdt(1,24,13+log2(8))  ConvertRealWorld=Stored Integer (SI)  SaturateOnIntegerOverflow=off  RndMeth=Floor
  Unit Delay Enabled Synchronous : hdlsllib/Discrete/Unit Delay Enabled Synchronous  InitialCondition=0.0  SampleTime=-1
  Unit Delay Enabled Resettable Synchronous : hdlsllib/Discrete/Unit Delay Enabled Resettable Synchronous  InitialCondition=0.0  SampleTime=-1
  avgEst : Outport
  wires:
  validIn/1 -> Delay1/1
  estin/1 -> Delay/1
  Data Type Conversion/1 -> Add/2
  Add/1 -> Data Type Conversion1/1
  Unit Delay Enabled Resettable Synchronous/1 -> Add/1, Divide by 8/1
  Data Type Conversion1/1 -> Unit Delay Enabled Resettable Synchronous/1
  Delay/1 -> Data Type Conversion/1
  Delay1/1 -> Unit Delay Enabled Resettable Synchronous/2
  endIn/1 -> Delay2/1
  Delay2/1 -> Delay3/1, Unit Delay Enabled Synchronous/2
  Delay3/1 -> Unit Delay Enabled Resettable Synchronous/3
  Divide by 8/1 -> Unit Delay Enabled Synchronous/1
  Unit Delay Enabled Synchronous/1 -> Data Type Conversion2/1
  Data Type Conversion2/1 -> avgEst/1

== system commhdlQPSKTxRxLoopback/Receiver/QPSK Rx/Frequency and Time Synchronizer/Phase Ambiguity Estimation and Correction/Phase Ambiguity Corrector ==
  note: Let Z be the complex Phase Ambiguity estimate and Xbar be the data and X be the corrected data.
      | X = Xbar * conj(Z) * (1/abs(Z))
  note: Set this value to zero to disable phase ambiguity correction
  dataIn : Inport
  estimate : Inport  Port=2
  validIn : Inport  Port=3
  Complex to Magnitude-Angle : dsphdlmathfun2/Complex to Magnitude-Angle  NumIterationsSource=Auto  NumIterations=10  OutputFormat=Magnitude  AngleFormat=Normalized  ScaleOutput=on  ScalingMethod=Shift-Add  SimulateUsing=Code generation
  Constant : Constant  OutDataTypeStr=boolean  SampleTime=-1
  Constant1 : Constant  OutMin=1  OutMax=1  OutDataTypeStr=boolean  SampleTime=-1
  Data Type Conversion : DataTypeConversion  OutDataTypeStr=fixdt(1,12,10)  SaturateOnIntegerOverflow=off  RndMeth=Floor
  Delay : Delay  DelayLength=15
  Delay1 : Delay  DelayLength=15
  Delay{2..4,7..8,10,13..18,22,25,28,36,38..39,41} (19 alike) : Delay  InitialCondition=0
  Delay11 : Delay  DelayLength=7  InitialCondition=0
  Delay12 : Delay  DelayLength=7  InitialCondition=0
  Delay5 : Delay  DelayLength=15
  Delay9 : Delay  DelayLength=7  InitialCondition=0
  Math Function : Math  Operator=conj  SignedPower=on  RndMeth=Zero
  Multiport Switch1 : MultiPortSwitch  DataPortOrder=Zero-based contiguous  Inputs=2  zeroidx=on  SaturateOnIntegerOverflow=off  InputSameDT=off
  Product1 : Product  OutDataTypeStr=Inherit: Same as first input
  Product2 : Product  OutDataTypeStr=Inherit: Same as first input
  Reciprocal : Subsystem  mask{WL=13, FL=10, outWL=26, Mapp=RAM - Based}
      mask prompts: WL "Input Word Length :"; FL "Input Fractional Length :"; outWL "Output Word Length :"; Mapp "Mapping Type:"
      mask init:
      | % Inverse for 18 bit numbers: partitioned into 3+15 bits. 2^3 LUTs with 2^15
      | % combinations will store a total of 2^18 combinations.
      | % As each LUT has 2^15 combinations the data type of output has a maximum
      | % limit of 32 bits (2^20 is a maximum number of bits an LUT can store)
      | 
      | % Non tunable Parameters
      | % FL = 16;
      | % outWL = 31;
      | % WL = 18;
      | % This Parameter is not given for mask
      | LUTAddrWL = WL - 1; % this will implement 2 LUTs
      | 
      | % validate Non tunable parameters
      | % condition for validation: 2^20 bits is the maximum number of bits an LUT can store
      | if LUTAddrWL >= 20   % As 2^20 is the limit
      |     error('invalid LUTAddrWL');
      | end
      | if outWL >= 2^(20-LUTAddrWL)  % 2^(20-LUTAddrWL) is the maximum outWL based on condition for validation
      |     error('invalid outWL')
      | end
      | 
      | % calculate number of LUTs required
      | muxSelectorWL = WL - LUTAddrWL;
      | nLUT = 2^muxSelectorWL;
      | 
      | % Generate all possible RWV inputs using WL and FL
      | allInputRangeSI = -2^(WL-1):2^(WL-1)-1;  % as a stored integer
      | allInputRWV = allInputRangeSI * 2^(-FL);
      | 
      | % define the function for all the RWV input
      | reciprocal = 1./allInputRWV;
      | 
      | % store the function output in LUT
      | allLUTAddr = (0:2^LUTAddrWL-1);
      | LUT = zeros(length(allLUTAddr),nLUT);
      | for i = 0:nLUT-1
      |     LUT(:,i+1) = reciprocal(i*2^LUTAddrWL+1:(i+1)*2^LUTAddrWL);
      | end
      | 
      | % quantize the function with outWL
      | NT = numerictype(fi(LUT(abs(LUT) ~= inf),1,outWL)); % inf and -inf will be quantized with max and min values with NT data type
      | if NT.WordLength < NT. FractionLength
      |     NT.FractionLength = NT.WordLength
      | end
      | LUT = fi(LUT,NT);
      | 
      | paths = find_system([gcb '/Function Impl'],'BlockType','Delay');
      | 
      | for i = 1:length(paths)
      |     if Mapp == 1
      |         hdlset_param(paths{i},'ResetType','default');
      |     else
      |         hdlset_param(paths{i},'ResetType','none');
      |     end
      | end
      mask TypeOptions Mapp: LUT - Based | RAM - Based
      mask DialogControl DescGroupVar Prompt: LUT - Based function
      mask DialogControl DescTextVar Prompt: This block is implemented for complex reciprocal
      mask Display: disp(['Reciprocal\n' get_param(gcb,'Mapp') '\nLatency = 7'])
  Terminator : Terminator
  dataOut : Outport
  validOut : Outport  Port=2
  wires:
  Delay3/1 -> Delay7/1
  Delay18/1 -> Delay22/1
  Delay17/1 -> Product1/2
  Delay15/1 -> Product1/1
  Delay13/1 -> Delay41/1
  Delay10/1 -> Reciprocal/1(dataIn)
  Delay12/1 -> Delay14/1
  Delay11/1 -> Delay36/1
  Delay9/1 -> Math Function/1
  Delay4/1 -> Delay15/1
  Delay41/1 -> Multiport Switch1/2
  Delay8/1 -> Delay11/1
  Delay/1 -> Delay8/1
  dataIn/1 -> Delay/1
  validIn/1 -> Delay5/1
  Delay5/1 -> Delay2/1
  Delay2/1 -> Delay12/1
  Delay14/1 -> Delay16/1
  Product2/1 -> Delay4/1
  Multiport Switch1/1 -> dataOut/1
  Delay22/1 -> validOut/1
  Constant/1 -> Multiport Switch1/1
  Delay16/1 -> Delay18/1
  Delay28/1 -> Product2/2
  Math Function/1 -> Delay28/1
  Delay25/1 -> Delay9/1
  Delay1/1 -> Delay25/1
  Delay36/1 -> Product2/1, Delay38/1
  Delay38/1 -> Delay13/1
  estimate/1 -> Data Type Conversion/1
  Reciprocal/1(dataOut) -> Delay3/1
  Product1/1 -> Delay39/1
  Constant1/1 -> Complex to Magnitude-Angle/2
  Complex to Magnitude-Angle/1 -> Delay10/1
  Complex to Magnitude-Angle/2 -> Terminator/1
  Delay39/1 -> Multiport Switch1/3
  Delay7/1 -> Delay17/1
  Data Type Conversion/1 -> Delay1/1, Complex to Magnitude-Angle/1

== system commhdlQPSKTxRxLoopback/Receiver/QPSK Rx/Frequency and Time Synchronizer/Phase Ambiguity Estimation and Correction/Phase Ambiguity Estimator ==
  dataIn : Inport
  syncPulse : Inport  Port=2
  validIn : Inport  Port=3
  Compare To Constant : simulink/Logic and Bit Operations/Compare To Constant  relop===  const=7  OutDataTypeStr=boolean
  Delay{1..3,8} (4 alike) : Delay  DelayLength=1
  Delay{4..7,9..11} (7 alike) : Delay
  Direct Lookup Table (n-D) : LookupNDDirect  NumberOfTableDimensions=1  Table=fi(preambleSymbols(3+1:3+8),1,16)  DiagnosticForOutOfRangeInput=Error
  HDL Counter : hdlsllib/Sources/HDL Counter  CountType=Count limited  CountInit=0  CountStep=1  CountMax=8-1  CountFromType=Initial value  CountFrom=0  CountResetPort=on  CountLoadPort=off  CountEnbPort=on  CountDirPort=off  CountHitOutputPort=off  CountDataType=Unsigned  CountWordLen=3  CountFracLen=0  CountSampTime=1
  Logical Operator : Logic  IconShape=distinctive  AllPortsSameDT=off  OutDataTypeStr=boolean
  Math Function : Math  Operator=conj  SignedPower=on  RndMeth=Zero
  Product : Product
  Subsystem : Subsystem
  Subsystem1 : Subsystem
  endOut : Outport
  estOut : Outport  Port=2
  validOut : Outport  Port=3
  wires:
  Compare To Constant/1 -> Logical Operator/2
  Subsystem/1(Out2) -> Subsystem1/1(In1), HDL Counter/1
  Direct Lookup Table (n-D)/1 -> Math Function/1
  Math Function/1 -> Delay4/1
  Product/1 -> Delay9/1
  Delay8/1 -> Direct Lookup Table (n-D)/1
  Delay1/1 -> Delay5/1
  Delay2/1 -> Delay6/1
  Delay3/1 -> Delay7/1
  Delay4/1 -> Product/2
  Delay5/1 -> Product/1
  Delay6/1 -> Delay10/1
  Delay7/1 -> Delay11/1
  Delay9/1 -> estOut/1
  Delay10/1 -> validOut/1
  Delay11/1 -> endOut/1
  dataIn/1 -> Delay1/1
  HDL Counter/1 -> Delay8/1, Compare To Constant/1
  Subsystem1/1(validOut) -> Delay2/1, Logical Operator/1, HDL Counter/2
  Logical Operator/1 -> Delay3/1, Subsystem/2(H)
  syncPulse/1 -> Subsystem/1(L)
  validIn/1 -> Subsystem1/2(validIn)

== system commhdlQPSKTxRxLoopback/Receiver/QPSK Rx/Frequency and Time Synchronizer/Preamble Detector/Correlator ==
  dataIn : Inport
  validIn : Inport  Port=2
  Complex to Real-Imag : ComplexToRealImag  Output=Real
  Delay{1..6} (6 alike) : Delay  DelayLength=1
  Delay7 : Delay  DelayLength=4
  Delay8 : Delay  DelayLength=4
  Discrete FIR Filter : dsphdlfiltering2/Discrete FIR Filter  NumeratorSource=Property  Numerator=rxPreambleMFCoeffs  NumeratorPrototype=[]  FilterStructure=Direct form systolic  SerializationOption=Minimum number of cycles between valid input samples  NumCycles=2  NumberOfMultipliers=2  SimulateUsing=Code generation  roundingMode=Floor  overflowMode=off  CoefficientsDataTypeStr=Inherit: Same word length as input  OutputDataTypeStr=Inherit: Same word length as input  ResetInputPort=off  HDLGlobalReset=off  CoeffMultiplier=Multiplier  UseMultForPow2Coeff=on  FrameInputSymmOptim=off
  Magnitude Squared : Subsystem
  Magnitude Squared and Moving Sum : Subsystem
  ThresholdLimiter : MATLAB Function  TreatAsAtomicUnit=on
  dataOut : Outport
  threshold : Outport  Port=2
  validOut : Outport  Port=3
  wires:
  Discrete FIR Filter/2 -> Delay1/1
  validIn/1 -> Magnitude Squared and Moving Sum/2(validIn), Discrete FIR Filter/2
  Discrete FIR Filter/1 -> Delay6/1
  Delay1/1 -> Delay7/1
  Delay3/1 -> validOut/1
  dataIn/1 -> Magnitude Squared and Moving Sum/1(scaled1), Discrete FIR Filter/1
  Delay4/1 -> ThresholdLimiter/1(x)
  Delay2/1 -> dataOut/1
  Delay5/1 -> threshold/1
  Magnitude Squared and Moving Sum/1(E1) -> Delay4/1
  Delay6/1 -> Magnitude Squared/1(In1)
  Magnitude Squared/1(Out1) -> Complex to Real-Imag/1
  ThresholdLimiter/1(y) -> Delay8/1
  Delay7/1 -> Delay3/1
  Delay8/1 -> Delay5/1
  Complex to Real-Imag/1 -> Delay2/1
